simulink model "pfb_fir_test"  (Simulink 7.2)
settings: Solver=VariableStepDiscrete  StartTime=0.0  StopTime=500  RelTol=1e-3
undefined symbols (not defined in the file or in its folder): pfb_coeff_gen_calc
libraries: xbsIndex_r4 x240, casper_library_delays x20, casper_library_misc x18
(part 1 of 4)
settings Model: Creator=User  LastModifiedBy=root
settings OptimizationCC: InitFltsAndDblsToZero=on
settings DebuggingCC: SaveWithDisabledLinksMsg=none  SaveWithParameterizedLinksMsg=none

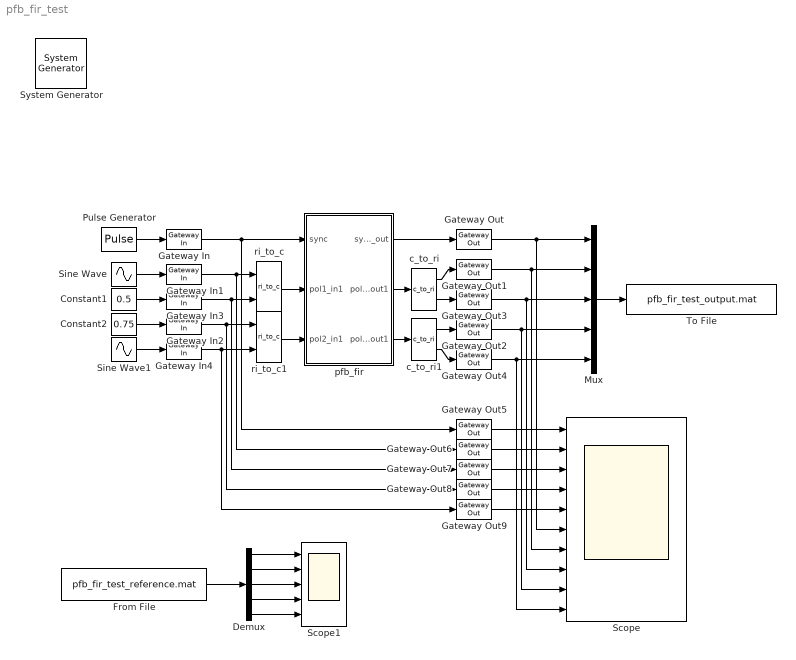
== system pfb_fir_test ==
  " System Generator" : xbsIndex_r4/ System Generator  Tag=genX  SystemSampleTime=-1  xilinxfamily=Virtex4  part=xc4vsx35  speed=-10  package=ff668  synthesis_tool=XST  clock_wrapper=Clock Enables  directory=./netlist  testbench=off  simulink_period=1  sysclk_period=100  dcm_input_clock_period=100  incr_netlist=off  trim_vbits=Everywhere in SubSystem  dbl_ovrd=According to Block Masks  core_generation=According to Block Masks  run_coregen=off  deprecated_control=off  eval_field=0  block_type=sysgen
      settings: block_version=10.1.1
  Constant1 : Constant  Value=0.5  OutDataType=sfix(16)  OutScaling=2^0
  Constant2 : Constant  Value=0.75  OutDataType=sfix(16)  OutScaling=2^0
  Demux : Demux  Outputs=5
  From File : FromFile  FileName=pfb_fir_test_reference.mat  SampleTime=1
  Gateway In : xbsIndex_r4/Gateway In  arith_type=Boolean  n_bits=16  bin_pt=14  quantization="Round  (unbiased: +/- Inf)"  overflow=Saturate  period=1  dbl_ovrd=off  timing_constraint=None  locs_specified=off  LOCs={}  hdl_port=on  block_type=gatewayin
      settings: infoedit="Gateway in block.  Converts inputs of type Simulink integer, double and fixed point to  Xilinx fixed point type.<P><P>Hardware notes:  In hardware these blocks become top level input ports."  block_version=10.1.1
  Gateway In{1..4} (4 alike) : xbsIndex_r4/Gateway In  arith_type="Signed  (2's comp)"  n_bits=12  bin_pt=11  quantization=Truncate  overflow=Wrap  period=1  dbl_ovrd=off  timing_constraint=None  locs_specified=off  LOCs={}  hdl_port=on  block_type=gatewayin
      settings: infoedit="Gateway in block.  Converts inputs of type Simulink integer, double and fixed point to  Xilinx fixed point type.<P><P>Hardware notes:  In hardware these blocks become top level input ports."  block_version=10.1.1
  Gateway Out{,1..9} (10 alike) : xbsIndex_r4/Gateway Out  hdl_port=on  timing_constraint=None  locs_specified=off  LOCs={}  block_type=gatewayout
      settings: infoedit="Gateway out block.  Converts Xilinx fixed point inputs into ouputs of type Simulink integer, double, or fixed point.<P><P>Hardware notes:  In hardware these blocks become top level output ports or are discarded, depending on how they are configured."  block_version=10.1.1
  Mux : Mux  Inputs=5
  Pulse Generator : DiscretePulseGenerator  Period=2^10  PhaseDelay=13
  Scope : Scope  NumInputPorts=10
      settings: YMin=-5~-5~-5~-5~-5~-5~-5~-5~-5~-5  YMax=5~5~5~5~5~5~5~5~5~5
  Scope1 : Scope  NumInputPorts=5
      settings: YMin=-5~-5~-5~-5~-5  YMax=5~5~5~5~5
  Sine Wave : Sin  SineType=Sample based  Amplitude=0.8  Samples=16  SampleTime=1  Offset=7
  Sine Wave1 : Sin  SineType=Sample based  Amplitude=0.8  Samples=8  SampleTime=1  Offset=7
  To File : ToFile  Filename=pfb_fir_test_output.mat  MatrixName=output
  c_to_ri : casper_library_misc/c_to_ri  SystemSampleTime=-1  n_bits=20  bin_pt=19
      settings: AttributesFormatString=20_19 r/i
  c_to_ri1 : casper_library_misc/c_to_ri  SystemSampleTime=-1  n_bits=20  bin_pt=19
      settings: AttributesFormatString=20_19 r/i
  pfb_fir : Subsystem  AncestorBlock=casper_library_pfbs/pfb_fir  mask(pfb_fir){PFBSize=6, TotalTaps=6, WindowType=nuttallwin, n_inputs=0, MakeBiplex=1, BitWidthIn=12, BitWidthOut=20, CoeffBitWidth=8, CoeffDistMem=1, add_latency=1, mult_latency=2, bram_latency=1, quantization=Round  (unbiased: +/- Inf), fwidth=0.75, specify_mult=off, mult_spec=[2                                      2]}
      mask prompts: PFBSize "Size of PFB: (2^? pnts)"; TotalTaps "Total Number of Taps:"; WindowType "Windowing Function:"; n_inputs "Number of Simultaneous Inputs: (2^?)"; MakeBiplex "Make Biplex"; BitWidthIn "Input Bitwidth:"; BitWidthOut "Output Bitwidth:"; CoeffBitWidth "Coefficient Bitwidth:"; CoeffDistMem "Use Distributed Memory for Coeffs"; add_latency "Add Latency"; mult_latency "Mult Latency"; bram_latency "BRAM Latency"; quantization "Quantization Behavior"; fwidth "Bin Width Scaling (normal=1)"; specify_mult "Specify multiplier use (behavioral if not specified)"; mult_spec "Multiplier specification (0=core, 1=embedded, 2=behavioural) (left=1st tap)"
      mask init:
      | pfb_fir_init(gcb, ...
      |     'PFBSize', PFBSize, ...
      |     'TotalTaps', TotalTaps, ...
      |     'WindowType', WindowType, ...
      |     'n_inputs', n_inputs, ...
      |     'MakeBiplex', MakeBiplex, ...
      |     'BitWidthIn', BitWidthIn, ...
      |     'BitWidthOut', BitWidthOut, ...
      |     'CoeffBitWidth', CoeffBitWidth, ...
      |     'CoeffDistMem', CoeffDistMem, ...
      |     'add_latency', add_latency, ...
      |     'mult_latency', mult_latency, ...
      |     'bram_latency', bram_latency, ...
      |     'quantization', quantization, ...
      |     'fwidth', fwidth,...
      |     'specify_mult', specify_mult,...
      |     'mult_spec', mult_spec);
      settings: AttributesFormatString=|
      | taps=6, add_latency=1
      | max scale 0.696
      mask Help: eval('xlWeb(''http://casper.berkeley.edu/wiki/Pfb_fir'')')
      mask StyleString: edit,edit,popup(bartlett|barthannwin|blackman|blackmanharris|bohamwin|chebwin|flattopwin|gausswin|hamming|hann|kaiser|nuttallwin|parzenwin|rectwin|tukeywin|triang|userwindow),edit,edit,edit,edit,edit,edit,edit,edit,edit,popup(Truncate|Round  (unbiased: +/- Inf)|Round  (unbiased: Even Values)),edit,checkbox,edit
      mask CallbackString:
      | |%num_taps = eval(get_param(gcb, 'TotalTaps'));
      | %old_vec = eval(get_param(gcb, 'mult_spec'));
      | 
      | %vec = 2.*ones(1,num_taps);
      | %old_size = length(old_vec);
      | 
      | %if(old_size <= num_taps),
      | %   new_size = old_size;
      | %else,
      | %    new_size = num_taps;
      | %end
      | 
      | %for n = 1:new_size, vec(n) = old_vec(n); end
      | %set_param(gcb, 'mult_spec', mat2str(vec));||||||||||||%num_taps = eval(get_param(gcb, 'TotalTaps'));
      | %old_vec = eval(get_param(gcb, 'mult_spec'));
      | 
      | %vec = 2.*ones(1,num_taps);
      | %old_size = length(old_vec);
      | 
      | %if(old_size <= num_taps),
      | %    new_size = old_size;
      | %else,
      | %    new_size = num_taps;
      | %end
      | 
      | %for n = 1:new_size, vec(n) = old_vec(n); end
      | %set_param(gcb, 'mult_spec', mat2str(vec));|%specify_mult = get_param(gcb,'specify_mult');
      | %if( strcmp(specify_mult,'off')),
      | %    set_param(gcb, 'MaskEnables', {'on','on','on','on','on','on','on','on','on','on','on','on','on','on','on','off'});
      | %else
      | %    set_param(gcb, 'MaskEnables', {'on','on','on','on','on','on','on','on','on','on','on','on','on','on','on','on'});
      | %end
      | 
      | |%specify_mult = get_param(gcb,'specify_mult');
      | %if( strcmp(specify_mult,'off')),
      | %    set_param(gcb, 'MaskEnables', {'on','on','on','on','on','on','on','on','on','on','on','on','on','on','on','off'});
      | %else
      | %    set_param(gcb, 'MaskEnables', {'on','on','on','on','on','on','on','on','on','on','on','on','on','on','on','on'});
      | %end
  ri_to_c : casper_library_misc/ri_to_c  SystemSampleTime=-1
  ri_to_c1 : casper_library_misc/ri_to_c  SystemSampleTime=-1
  wires:
  Pulse Generator/1 -> Gateway In/1
  Gateway In/1 -> Gateway Out5/1, pfb_fir/1(sync)
  Sine Wave/1 -> Gateway In1/1
  Constant2/1 -> Gateway In2/1
  pfb_fir/1(sync_out) -> Gateway Out/1
  Constant1/1 -> Gateway In3/1
  Sine Wave1/1 -> Gateway In4/1
  Gateway In1/1 -> ri_to_c/1, Gateway Out6/1
  Gateway In3/1 -> ri_to_c/2, Gateway Out7/1
  Gateway In2/1 -> ri_to_c1/1, Gateway Out8/1
  Gateway In4/1 -> ri_to_c1/2, Gateway Out9/1
  ri_to_c/1 -> pfb_fir/2(pol1_in1)
  ri_to_c1/1 -> pfb_fir/3(pol2_in1)
  pfb_fir/2(pol1_out1) -> c_to_ri/1
  c_to_ri/1 -> Gateway Out1/1
  c_to_ri/2 -> Gateway Out3/1
  pfb_fir/3(pol2_out1) -> c_to_ri1/1
  c_to_ri1/1 -> Gateway Out2/1
  c_to_ri1/2 -> Gateway Out4/1
  Gateway Out5/1 -> Scope/1
  Gateway Out6/1 -> Scope/2
  Gateway Out7/1 -> Scope/3
  Gateway Out8/1 -> Scope/4
  Gateway Out9/1 -> Scope/5
  Gateway Out/1 -> Scope/6, Mux/1
  Gateway Out1/1 -> Scope/7, Mux/2
  Gateway Out3/1 -> Scope/8, Mux/3
  Gateway Out2/1 -> Scope/9, Mux/4
  Gateway Out4/1 -> Scope/10, Mux/5
  Mux/1 -> To File/1
  From File/1 -> Demux/1
  Demux/1 -> Scope1/1
  Demux/2 -> Scope1/2
  Demux/3 -> Scope1/3
  Demux/4 -> Scope1/4
  Demux/5 -> Scope1/5

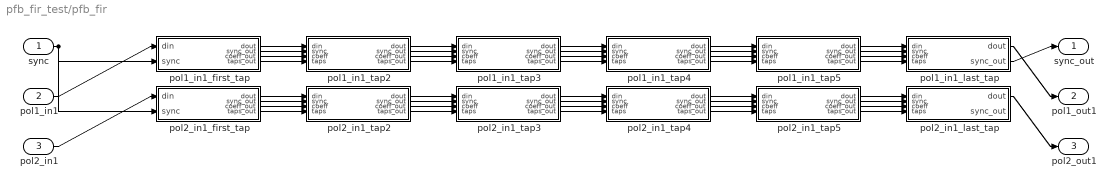
== system pfb_fir_test/pfb_fir ==
  sync : Inport
  pol1_in1 : Inport  Port=2
  pol2_in1 : Inport  Port=3
  pol1_in1_first_tap : Subsystem  AncestorBlock=casper_library_pfbs/first_tap  mask(first_tap){nput=0, PFBSize=6, CoeffBitWidth=8, TotalTaps=6, BitWidthIn=12, CoeffDistMem=1, WindowType=nuttallwin, mult_latency=2, bram_latency=1, n_inputs=0, fwidth=0.75, use_hdl=on, use_embedded=off}
      mask prompts: nput "This is input number:"; PFBSize "Size of PFB: (2^? pnts)"; CoeffBitWidth "Bitwidth of Coefficients:"; TotalTaps "Total Number of Taps:"; BitWidthIn "Input Bitwidth:"; CoeffDistMem "Implement Coeff Gen in Distributed Memory:"; WindowType "Windowing Function:"; mult_latency "Mult Latency"; bram_latency "BRAM Latency"; n_inputs "Number of Simultaneous Inputs: (2^?)"; fwidth "Bit Width (normal=1)"; use_hdl "Use behavioral HDL for multlipliers"; use_embedded "Use embedded multipliers"
      mask init:
      | first_tap_init(gcb,...
      |     'nput', nput,...
      |     'PFBSize', PFBSize,...
      |     'CoeffBitWidth', CoeffBitWidth,...
      |     'TotalTaps', TotalTaps,...
      |     'BitWidthIn', BitWidthIn,...
      |     'CoeffDistMem', CoeffDistMem,...
      |     'WindowType', WindowType,...
      |     'mult_latency', mult_latency,...
      |     'bram_latency', bram_latency,...
      |     'n_inputs', n_inputs,...
      |     'fwidth', fwidth,...
      |     'use_hdl', use_hdl,...
      |     'use_embedded', use_embedded);
      settings: AttributesFormatString=input=0, taps=6
      mask StyleString: edit,edit,edit,edit,edit,edit,popup(bartlett|barthannwin|blackman|blackmanharris|bohamwin|chebwin|flattopwin|gausswin|hamming|hann|kaiser|nuttallwin|parzenwin|rectwin|tukeywin|triang),edit,edit,edit,edit,checkbox,checkbox
      mask CallbackString:
      | |||||||||||use_hdl = get_param(gcb,'use_hdl');
      | if( strcmp(use_hdl,'on')),
      |     set_param(gcb, 'use_embedded','off');
      |     set_param(gcb, 'MaskVisibilities',{'on','on','on','on','on','on','on','on','on','on','on','on','off'});
      | else,
      |     set_param(gcb, 'MaskVisibilities',{'on','on','on','on','on','on','on','on','on','on','on','on','on'});
      | end
      | |
  pol1_in1_last_tap : Subsystem  AncestorBlock=casper_library_pfbs/last_tap  mask(last_tap){TotalTaps=6, BitWidthIn=12, BitWidthOut=20, CoeffBitWidth=8, add_latency=1, mult_latency=2, quantization=Round  (unbiased: +/- Inf), use_hdl=on, use_embedded=off}
      mask prompts: TotalTaps "Total Number of Taps:"; BitWidthIn "Input Bitwidth:"; BitWidthOut "Output Bitwidth:"; CoeffBitWidth "Coeff Bitwidth:"; add_latency "Add Latency"; mult_latency "Mult Latency"; quantization "Quantization Behavior"; use_hdl "Use behavioral HDL for multlipliers"; use_embedded "Use embedded multipliers"
      mask init:
      | last_tap_init(gcb,...
      |     'TotalTaps', TotalTaps,...
      |     'BitWidthIn', BitWidthIn,...
      |     'BitWidthOut', BitWidthOut,...
      |     'CoeffBitWidth', CoeffBitWidth,...
      |     'add_latency', add_latency,...
      |     'mult_latency', mult_latency,...
      |     'quantization', quantization,...
      |     'use_hdl', use_hdl,...
      |     'use_embedded', use_embedded);
      settings: AttributesFormatString=taps=6
      mask StyleString: edit,edit,edit,edit,edit,edit,popup(Truncate|Round  (unbiased: +/- Inf)|Round  (unbiased: Even Values)),checkbox,checkbox
      mask CallbackString:
      | |||||||use_hdl = get_param(gcb,'use_hdl');
      | if( strcmp(use_hdl,'on')),
      |     set_param(gcb, 'use_embedded','off');
      |     set_param(gcb, 'MaskVisibilities',{'on','on','on','on','on','on','on','on','off'});
      | else,
      |     set_param(gcb, 'MaskVisibilities',{'on','on','on','on','on','on','on','on','on'});
      | end
      | |
  pol1_in1_tap2 : Subsystem  AncestorBlock=casper_library_pfbs/tap  mask(tap){mult_latency=2, coeff_width=8, coeff_frac_width=7, delay=64, data_width=12, bram_latency=1, use_hdl=on, use_embedded=off}
      mask prompts: mult_latency "Multiplier Latency"; coeff_width "Coefficient Bit Width In"; coeff_frac_width "Coefficient Fractional Bits"; delay "Data/Sync Delay"; data_width "Data Bit Width In"; bram_latency "BRAM Latency"; use_hdl "Use behavioral HDL for multlipliers"; use_embedded "Use embedded multipliers"
      mask init:
      | use_hdl = get_param(gcb,'use_hdl');
      | use_embedded = get_param(gcb,'use_embedded');
      | set_param(gcb,'LinkStatus','inactive');
      | 
      | set_param([gcb,'/Mult'],'use_embedded',use_embedded);
      | set_param([gcb,'/Mult'],'use_behavioral_HDL',use_hdl);
      | set_param([gcb,'/Mult1'],'use_embedded',use_embedded);
      | set_param([gcb,'/Mult1'],'use_behavioral_HDL',use_hdl);
      mask CallbackString:
      | ||||||use_hdl = get_param(gcb,'use_hdl');
      | if( strcmp(use_hdl,'on')),
      |     set_param(gcb, 'use_embedded','off');
      |     set_param(gcb, 'MaskVisibilities',{'on','on','on','on','on','on','on','off'});
      | else,
      |     set_param(gcb, 'MaskVisibilities',{'on','on','on','on','on','on','on','on'});
      | end
      | |
  pol1_in1_tap3 : Subsystem  AncestorBlock=casper_library_pfbs/tap  mask(tap){mult_latency=2, coeff_width=8, coeff_frac_width=7, delay=64, data_width=12, bram_latency=1, use_hdl=on, use_embedded=off}
      mask prompts: mult_latency "Multiplier Latency"; coeff_width "Coefficient Bit Width In"; coeff_frac_width "Coefficient Fractional Bits"; delay "Data/Sync Delay"; data_width "Data Bit Width In"; bram_latency "BRAM Latency"; use_hdl "Use behavioral HDL for multlipliers"; use_embedded "Use embedded multipliers"
      mask init: same as pfb_fir_test/pfb_fir/pol1_in1_tap2
      mask CallbackString:
      | ||||||use_hdl = get_param(gcb,'use_hdl');
      | if( strcmp(use_hdl,'on')),
      |     set_param(gcb, 'use_embedded','off');
      |     set_param(gcb, 'MaskVisibilities',{'on','on','on','on','on','on','on','off'});
      | else,
      |     set_param(gcb, 'MaskVisibilities',{'on','on','on','on','on','on','on','on'});
      | end
      | |
  pol1_in1_tap4 : Subsystem  AncestorBlock=casper_library_pfbs/tap  mask(tap){mult_latency=2, coeff_width=8, coeff_frac_width=7, delay=64, data_width=12, bram_latency=1, use_hdl=on, use_embedded=off}
      mask prompts: mult_latency "Multiplier Latency"; coeff_width "Coefficient Bit Width In"; coeff_frac_width "Coefficient Fractional Bits"; delay "Data/Sync Delay"; data_width "Data Bit Width In"; bram_latency "BRAM Latency"; use_hdl "Use behavioral HDL for multlipliers"; use_embedded "Use embedded multipliers"
      mask init: same as pfb_fir_test/pfb_fir/pol1_in1_tap2
      mask CallbackString:
      | ||||||use_hdl = get_param(gcb,'use_hdl');
      | if( strcmp(use_hdl,'on')),
      |     set_param(gcb, 'use_embedded','off');
      |     set_param(gcb, 'MaskVisibilities',{'on','on','on','on','on','on','on','off'});
      | else,
      |     set_param(gcb, 'MaskVisibilities',{'on','on','on','on','on','on','on','on'});
      | end
      | |
  pol1_in1_tap5 : Subsystem  AncestorBlock=casper_library_pfbs/tap  mask(tap){mult_latency=2, coeff_width=8, coeff_frac_width=7, delay=64, data_width=12, bram_latency=1, use_hdl=on, use_embedded=off}
      mask prompts: mult_latency "Multiplier Latency"; coeff_width "Coefficient Bit Width In"; coeff_frac_width "Coefficient Fractional Bits"; delay "Data/Sync Delay"; data_width "Data Bit Width In"; bram_latency "BRAM Latency"; use_hdl "Use behavioral HDL for multlipliers"; use_embedded "Use embedded multipliers"
      mask init: same as pfb_fir_test/pfb_fir/pol1_in1_tap2
      mask CallbackString:
      | ||||||use_hdl = get_param(gcb,'use_hdl');
      | if( strcmp(use_hdl,'on')),
      |     set_param(gcb, 'use_embedded','off');
      |     set_param(gcb, 'MaskVisibilities',{'on','on','on','on','on','on','on','off'});
      | else,
      |     set_param(gcb, 'MaskVisibilities',{'on','on','on','on','on','on','on','on'});
      | end
      | |
  pol2_in1_first_tap : Subsystem  AncestorBlock=casper_library_pfbs/first_tap  mask(first_tap){nput=0, PFBSize=6, CoeffBitWidth=8, TotalTaps=6, BitWidthIn=12, CoeffDistMem=1, WindowType=nuttallwin, mult_latency=2, bram_latency=1, n_inputs=0, fwidth=0.75, use_hdl=on, use_embedded=off}
      mask prompts: nput "This is input number:"; PFBSize "Size of PFB: (2^? pnts)"; CoeffBitWidth "Bitwidth of Coefficients:"; TotalTaps "Total Number of Taps:"; BitWidthIn "Input Bitwidth:"; CoeffDistMem "Implement Coeff Gen in Distributed Memory:"; WindowType "Windowing Function:"; mult_latency "Mult Latency"; bram_latency "BRAM Latency"; n_inputs "Number of Simultaneous Inputs: (2^?)"; fwidth "Bit Width (normal=1)"; use_hdl "Use behavioral HDL for multlipliers"; use_embedded "Use embedded multipliers"
      mask init: same as pfb_fir_test/pfb_fir/pol1_in1_first_tap
      settings: AttributesFormatString=input=0, taps=6
      mask StyleString: edit,edit,edit,edit,edit,edit,popup(bartlett|barthannwin|blackman|blackmanharris|bohamwin|chebwin|flattopwin|gausswin|hamming|hann|kaiser|nuttallwin|parzenwin|rectwin|tukeywin|triang),edit,edit,edit,edit,checkbox,checkbox
      mask CallbackString:
      | |||||||||||use_hdl = get_param(gcb,'use_hdl');
      | if( strcmp(use_hdl,'on')),
      |     set_param(gcb, 'use_embedded','off');
      |     set_param(gcb, 'MaskVisibilities',{'on','on','on','on','on','on','on','on','on','on','on','on','off'});
      | else,
      |     set_param(gcb, 'MaskVisibilities',{'on','on','on','on','on','on','on','on','on','on','on','on','on'});
      | end
      | |
  pol2_in1_last_tap : Subsystem  AncestorBlock=casper_library_pfbs/last_tap  mask(last_tap){TotalTaps=6, BitWidthIn=12, BitWidthOut=20, CoeffBitWidth=8, add_latency=1, mult_latency=2, quantization=Round  (unbiased: +/- Inf), use_hdl=on, use_embedded=off}
      mask prompts: TotalTaps "Total Number of Taps:"; BitWidthIn "Input Bitwidth:"; BitWidthOut "Output Bitwidth:"; CoeffBitWidth "Coeff Bitwidth:"; add_latency "Add Latency"; mult_latency "Mult Latency"; quantization "Quantization Behavior"; use_hdl "Use behavioral HDL for multlipliers"; use_embedded "Use embedded multipliers"
      mask init: same as pfb_fir_test/pfb_fir/pol1_in1_last_tap
      settings: AttributesFormatString=taps=6
      mask StyleString: edit,edit,edit,edit,edit,edit,popup(Truncate|Round  (unbiased: +/- Inf)|Round  (unbiased: Even Values)),checkbox,checkbox
      mask CallbackString:
      | |||||||use_hdl = get_param(gcb,'use_hdl');
      | if( strcmp(use_hdl,'on')),
      |     set_param(gcb, 'use_embedded','off');
      |     set_param(gcb, 'MaskVisibilities',{'on','on','on','on','on','on','on','on','off'});
      | else,
      |     set_param(gcb, 'MaskVisibilities',{'on','on','on','on','on','on','on','on','on'});
      | end
      | |
  pol2_in1_tap2 : Subsystem  AncestorBlock=casper_library_pfbs/tap  mask(tap){mult_latency=2, coeff_width=8, coeff_frac_width=7, delay=64, data_width=12, bram_latency=1, use_hdl=on, use_embedded=off}
      mask prompts: mult_latency "Multiplier Latency"; coeff_width "Coefficient Bit Width In"; coeff_frac_width "Coefficient Fractional Bits"; delay "Data/Sync Delay"; data_width "Data Bit Width In"; bram_latency "BRAM Latency"; use_hdl "Use behavioral HDL for multlipliers"; use_embedded "Use embedded multipliers"
      mask init: same as pfb_fir_test/pfb_fir/pol1_in1_tap2
      mask CallbackString:
      | ||||||use_hdl = get_param(gcb,'use_hdl');
      | if( strcmp(use_hdl,'on')),
      |     set_param(gcb, 'use_embedded','off');
      |     set_param(gcb, 'MaskVisibilities',{'on','on','on','on','on','on','on','off'});
      | else,
      |     set_param(gcb, 'MaskVisibilities',{'on','on','on','on','on','on','on','on'});
      | end
      | |
  pol2_in1_tap3 : Subsystem  AncestorBlock=casper_library_pfbs/tap  mask(tap){mult_latency=2, coeff_width=8, coeff_frac_width=7, delay=64, data_width=12, bram_latency=1, use_hdl=on, use_embedded=off}
      mask prompts: mult_latency "Multiplier Latency"; coeff_width "Coefficient Bit Width In"; coeff_frac_width "Coefficient Fractional Bits"; delay "Data/Sync Delay"; data_width "Data Bit Width In"; bram_latency "BRAM Latency"; use_hdl "Use behavioral HDL for multlipliers"; use_embedded "Use embedded multipliers"
      mask init: same as pfb_fir_test/pfb_fir/pol1_in1_tap2
      mask CallbackString:
      | ||||||use_hdl = get_param(gcb,'use_hdl');
      | if( strcmp(use_hdl,'on')),
      |     set_param(gcb, 'use_embedded','off');
      |     set_param(gcb, 'MaskVisibilities',{'on','on','on','on','on','on','on','off'});
      | else,
      |     set_param(gcb, 'MaskVisibilities',{'on','on','on','on','on','on','on','on'});
      | end
      | |
  pol2_in1_tap4 : Subsystem  AncestorBlock=casper_library_pfbs/tap  mask(tap){mult_latency=2, coeff_width=8, coeff_frac_width=7, delay=64, data_width=12, bram_latency=1, use_hdl=on, use_embedded=off}
      mask prompts: mult_latency "Multiplier Latency"; coeff_width "Coefficient Bit Width In"; coeff_frac_width "Coefficient Fractional Bits"; delay "Data/Sync Delay"; data_width "Data Bit Width In"; bram_latency "BRAM Latency"; use_hdl "Use behavioral HDL for multlipliers"; use_embedded "Use embedded multipliers"
      mask init: same as pfb_fir_test/pfb_fir/pol1_in1_tap2
      mask CallbackString:
      | ||||||use_hdl = get_param(gcb,'use_hdl');
      | if( strcmp(use_hdl,'on')),
      |     set_param(gcb, 'use_embedded','off');
      |     set_param(gcb, 'MaskVisibilities',{'on','on','on','on','on','on','on','off'});
      | else,
      |     set_param(gcb, 'MaskVisibilities',{'on','on','on','on','on','on','on','on'});
      | end
      | |
  pol2_in1_tap5 : Subsystem  AncestorBlock=casper_library_pfbs/tap  mask(tap){mult_latency=2, coeff_width=8, coeff_frac_width=7, delay=64, data_width=12, bram_latency=1, use_hdl=on, use_embedded=off}
      mask prompts: mult_latency "Multiplier Latency"; coeff_width "Coefficient Bit Width In"; coeff_frac_width "Coefficient Fractional Bits"; delay "Data/Sync Delay"; data_width "Data Bit Width In"; bram_latency "BRAM Latency"; use_hdl "Use behavioral HDL for multlipliers"; use_embedded "Use embedded multipliers"
      mask init: same as pfb_fir_test/pfb_fir/pol1_in1_tap2
      mask CallbackString:
      | ||||||use_hdl = get_param(gcb,'use_hdl');
      | if( strcmp(use_hdl,'on')),
      |     set_param(gcb, 'use_embedded','off');
      |     set_param(gcb, 'MaskVisibilities',{'on','on','on','on','on','on','on','off'});
      | else,
      |     set_param(gcb, 'MaskVisibilities',{'on','on','on','on','on','on','on','on'});
      | end
      | |
  sync_out : Outport
  pol1_out1 : Outport  Port=2
  pol2_out1 : Outport  Port=3
  wires:
  pol1_in1/1 -> pol1_in1_first_tap/1(din)
  sync/1 -> pol1_in1_first_tap/2(sync), pol2_in1_first_tap/2(sync)
  pol1_in1_first_tap/1(dout) -> pol1_in1_tap2/1(din)
  pol1_in1_first_tap/2(sync_out) -> pol1_in1_tap2/2(sync)
  pol1_in1_first_tap/3(coeff_out) -> pol1_in1_tap2/3(coeff)
  pol1_in1_first_tap/4(taps_out) -> pol1_in1_tap2/4(taps)
  pol1_in1_tap2/1(dout) -> pol1_in1_tap3/1(din)
  pol1_in1_tap2/2(sync_out) -> pol1_in1_tap3/2(sync)
  pol1_in1_tap2/3(coeff_out) -> pol1_in1_tap3/3(coeff)
  pol1_in1_tap2/4(taps_out) -> pol1_in1_tap3/4(taps)
  pol1_in1_tap3/1(dout) -> pol1_in1_tap4/1(din)
  pol1_in1_tap3/2(sync_out) -> pol1_in1_tap4/2(sync)
  pol1_in1_tap3/3(coeff_out) -> pol1_in1_tap4/3(coeff)
  pol1_in1_tap3/4(taps_out) -> pol1_in1_tap4/4(taps)
  pol1_in1_tap4/1(dout) -> pol1_in1_tap5/1(din)
  pol1_in1_tap4/2(sync_out) -> pol1_in1_tap5/2(sync)
  pol1_in1_tap4/3(coeff_out) -> pol1_in1_tap5/3(coeff)
  pol1_in1_tap4/4(taps_out) -> pol1_in1_tap5/4(taps)
  pol1_in1_tap5/1(dout) -> pol1_in1_last_tap/1(din)
  pol1_in1_tap5/2(sync_out) -> pol1_in1_last_tap/2(sync)
  pol1_in1_tap5/3(coeff_out) -> pol1_in1_last_tap/3(coeff)
  pol1_in1_tap5/4(taps_out) -> pol1_in1_last_tap/4(taps)
  pol1_in1_last_tap/1(dout) -> pol1_out1/1
  pol1_in1_last_tap/2(sync_out) -> sync_out/1
  pol2_in1/1 -> pol2_in1_first_tap/1(din)
  pol2_in1_first_tap/1(dout) -> pol2_in1_tap2/1(din)
  pol2_in1_first_tap/2(sync_out) -> pol2_in1_tap2/2(sync)
  pol2_in1_first_tap/3(coeff_out) -> pol2_in1_tap2/3(coeff)
  pol2_in1_first_tap/4(taps_out) -> pol2_in1_tap2/4(taps)
  pol2_in1_tap2/1(dout) -> pol2_in1_tap3/1(din)
  pol2_in1_tap2/2(sync_out) -> pol2_in1_tap3/2(sync)
  pol2_in1_tap2/3(coeff_out) -> pol2_in1_tap3/3(coeff)
  pol2_in1_tap2/4(taps_out) -> pol2_in1_tap3/4(taps)
  pol2_in1_tap3/1(dout) -> pol2_in1_tap4/1(din)
  pol2_in1_tap3/2(sync_out) -> pol2_in1_tap4/2(sync)
  pol2_in1_tap3/3(coeff_out) -> pol2_in1_tap4/3(coeff)
  pol2_in1_tap3/4(taps_out) -> pol2_in1_tap4/4(taps)
  pol2_in1_tap4/1(dout) -> pol2_in1_tap5/1(din)
  pol2_in1_tap4/2(sync_out) -> pol2_in1_tap5/2(sync)
  pol2_in1_tap4/3(coeff_out) -> pol2_in1_tap5/3(coeff)
  pol2_in1_tap4/4(taps_out) -> pol2_in1_tap5/4(taps)
  pol2_in1_tap5/1(dout) -> pol2_in1_last_tap/1(din)
  pol2_in1_tap5/2(sync_out) -> pol2_in1_last_tap/2(sync)
  pol2_in1_tap5/3(coeff_out) -> pol2_in1_last_tap/3(coeff)
  pol2_in1_tap5/4(taps_out) -> pol2_in1_last_tap/4(taps)
  pol2_in1_last_tap/1(dout) -> pol2_out1/1

== system pfb_fir_test/pfb_fir/pol1_in1_first_tap ==
  din : Inport  OutDataType=sfix(16)  OutScaling=2^0
  sync : Inport  Port=2  OutDataType=sfix(16)  OutScaling=2^0
  Mult : xbsIndex_r4/Mult  precision=Full  arith_type="Signed  (2's comp)"  n_bits=8  bin_pt=2  quantization=Truncate  overflow=Wrap  en=off  latency=mult_latency  dbl_ovrd=off  use_behavioral_HDL=on  opt=Speed  use_embedded=off  optimum_pipeline=off  pipeline=on  use_rpm=on  placement_style=Rectangular shape  block_type=mult
      settings: infoedit=Hardware notes: To use the internal pipeline stage of the dedicated multiplier you must select 'Pipeline for maximum performance'.  xl_area=[0, 0, 0, 0, 0, 0, 0]  block_version=9.1.01
  Mult1 : xbsIndex_r4/Mult  precision=Full  arith_type="Signed  (2's comp)"  n_bits=8  bin_pt=2  quantization=Truncate  overflow=Wrap  en=off  latency=mult_latency  dbl_ovrd=off  use_behavioral_HDL=on  opt=Speed  use_embedded=off  optimum_pipeline=off  pipeline=on  use_rpm=on  placement_style=Rectangular shape  block_type=mult
      settings: infoedit=Hardware notes: To use the internal pipeline stage of the dedicated multiplier you must select 'Pipeline for maximum performance'.  xl_area=[0, 0, 0, 0, 0, 0, 0]  block_version=9.1.01
  Reinterpret : xbsIndex_r4/Reinterpret  force_arith_type=on  arith_type="Signed  (2's comp)"  force_bin_pt=on  bin_pt=CoeffBitWidth - 1  block_type=reinterpret
      settings: infoedit="Changes signal type without altering the binary representation.   You can changed the signal between signed and unsigned, and relocate the binary point.<P><P>Hardware notes: In hardware this block costs nothing.<P><P>Example:  Suppose the input is 6 bits wide, signed, with 2 fractional bits, and the output is forced to unsigned with 0 fractional bits.  Then an input of -2.0 (1110.00 in binary 2's complement) becomes an output of 56 (111000 in binary)."  block_version=9.1.01
  Slice : xbsIndex_r4/Slice  nbits=CoeffBitWidth  boolean_output=off  mode=Lower Bit Location + Width  bit1=0  base1=MSB of Input  bit0=0  base0=LSB of Input  dbl_ovrd=off  block_type=slice
      settings: infoedit="Extracts a given range of bits from each input sample and presents it at the output.  The output type is ordinarily unsigned with binary point at zero, but can be Boolean when the slice is one bit wide.<P><P>Hardware notes: In hardware this block costs nothing."  block_version=9.1.01
  Slice1 : xbsIndex_r4/Slice  nbits=CoeffBitWidth * (TotalTaps - 1)  boolean_output=off  mode=Two Bit Locations  bit1=0  base1=MSB of Input  bit0=CoeffBitWidth  base0=LSB of Input  dbl_ovrd=off  block_type=slice
      settings: infoedit="Extracts a given range of bits from each input sample and presents it at the output.  The output type is ordinarily unsigned with binary point at zero, but can be Boolean when the slice is one bit wide.<P><P>Hardware notes: In hardware this block costs nothing."  block_version=9.1.01
  c_to_ri : casper_library_misc/c_to_ri  SystemSampleTime=-1  n_bits=BitWidthIn  bin_pt=BitWidthIn-1
      settings: AttributesFormatString=12_11 r/i
  delay_bram : casper_library_delays/delay_bram  SystemSampleTime=-1  DelayLen=2^(PFBSize-n_inputs)  bram_latency=bram_latency  use_dsp48=off
  pfb_coeff_gen : Subsystem  AncestorBlock=casper_library_pfbs/pfb_coeff_gen  mask(pfb_coeff_gen){PFBSize=6, CoeffBitWidth=8, TotalTaps=6, CoeffDistMem=1, WindowType=nuttallwin, bram_latency=1, n_inputs=0, nput=0, fwidth=0.75}
      mask prompts: PFBSize "Size of PFB: (2^? pnts)"; CoeffBitWidth "Bitwidth of Coefficients:"; TotalTaps "Total Number of Taps:"; CoeffDistMem "Implement Coeff Gen in Distributed Memory"; WindowType "Windowing Function:"; bram_latency "BRAM Latency"; n_inputs "Number of Simultaneous Inputs: (2^?)"; nput "This is input number:"; fwidth "Bin Width (normal=1)"
      mask init:
      | pfb_coeff_gen_init(gcb, ...
      |     'PFBSize', PFBSize, ...
      |     'CoeffBitWidth', CoeffBitWidth, ...
      |     'TotalTaps', TotalTaps, ...
      |     'CoeffDistMem', CoeffDistMem, ...
      |     'WindowType', WindowType, ...
      |     'bram_latency', bram_latency, ...
      |     'n_inputs', n_inputs, ...
      |     'nput', nput, ...
      |     'fwidth', fwidth);
      settings: AttributesFormatString=PFBSize=6, n_inputs=0, taps=6
  ri_to_c : Subsystem
  sync_delay : casper_library_delays/sync_delay  SystemSampleTime=-1  DelayLen=2^(PFBSize-n_inputs)
  dout : Outport  OutDataType=sfix(16)  OutScaling=2^0
  sync_out : Outport  Port=2  OutDataType=sfix(16)  OutScaling=2^0
  coeff_out : Outport  Port=3  OutDataType=sfix(16)  OutScaling=2^0
  taps_out : Outport  Port=4  OutDataType=sfix(16)  OutScaling=2^0
  wires:
  ri_to_c/1(c) -> taps_out/1
  Mult/1 -> ri_to_c/2(im)
  Mult1/1 -> ri_to_c/1(re)
  c_to_ri/2 -> Mult/1
  c_to_ri/1 -> Mult1/1
  pfb_coeff_gen/3(coeff) -> Slice1/1, Slice/1
  pfb_coeff_gen/2(sync_out) -> sync_delay/1
  sync/1 -> pfb_coeff_gen/2(sync)
  pfb_coeff_gen/1(dout) -> delay_bram/1, c_to_ri/1
  din/1 -> pfb_coeff_gen/1(din)
  delay_bram/1 -> dout/1
  sync_delay/1 -> sync_out/1
  Slice1/1 -> coeff_out/1
  Slice/1 -> Reinterpret/1
  Reinterpret/1 -> Mult1/2, Mult/2

== system pfb_fir_test/pfb_fir/pol1_in1_last_tap ==
  din : Inport  OutDataType=sfix(16)  OutScaling=2^0
  sync : Inport  Port=2  OutDataType=sfix(16)  OutScaling=2^0
  coeff : Inport  Port=3  OutDataType=sfix(16)  OutScaling=2^0
  taps : Inport  Port=4  OutDataType=sfix(16)  OutScaling=2^0
  Concat : xbsIndex_r4/Concat  num_inputs=2  dbl_ovrd=off  block_type=concat
      settings: block_version=9.1.01
  Delay : xbsIndex_r4/Delay  en=off  latency=mult_latency  dbl_ovrd=off  reg_retiming=off  block_type=delay
      settings: xl_area=[0, 0, 0, 0, 0, 0, 0]  block_version=9.1.01
  Mult : xbsIndex_r4/Mult  precision=Full  arith_type="Signed  (2's comp)"  n_bits=8  bin_pt=2  quantization=Truncate  overflow=Wrap  en=off  latency=mult_latency  dbl_ovrd=off  use_behavioral_HDL=on  opt=Speed  use_embedded=off  optimum_pipeline=off  pipeline=on  use_rpm=on  placement_style=Rectangular shape  block_type=mult
      settings: infoedit=Hardware notes: To use the internal pipeline stage of the dedicated multiplier you must select 'Pipeline for maximum performance'.  xl_area=[0, 0, 0, 0, 0, 0, 0]  block_version=9.1.01
  Mult1 : xbsIndex_r4/Mult  precision=Full  arith_type="Signed  (2's comp)"  n_bits=8  bin_pt=2  quantization=Truncate  overflow=Wrap  en=off  latency=mult_latency  dbl_ovrd=off  use_behavioral_HDL=on  opt=Speed  use_embedded=off  optimum_pipeline=off  pipeline=on  use_rpm=on  placement_style=Rectangular shape  block_type=mult
      settings: infoedit=Hardware notes: To use the internal pipeline stage of the dedicated multiplier you must select 'Pipeline for maximum performance'.  xl_area=[0, 0, 0, 0, 0, 0, 0]  block_version=9.1.01
  Reinterpret : xbsIndex_r4/Reinterpret  force_arith_type=on  arith_type="Signed  (2's comp)"  force_bin_pt=on  bin_pt=CoeffBitWidth - 1  block_type=reinterpret
      settings: infoedit="Changes signal type without altering the binary representation.   You can changed the signal between signed and unsigned, and relocate the binary point.<P><P>Hardware notes: In hardware this block costs nothing.<P><P>Example:  Suppose the input is 6 bits wide, signed, with 2 fractional bits, and the output is forced to unsigned with 0 fractional bits.  Then an input of -2.0 (1110.00 in binary 2's complement) becomes an output of 56 (111000 in binary)."  block_version=9.1.01
  c_to_ri : casper_library_misc/c_to_ri  SystemSampleTime=-1  n_bits=BitWidthIn  bin_pt=BitWidthIn-1
      settings: AttributesFormatString=12_11 r/i
  pfb_add_tree : Subsystem  mask(pfb_add_tree){TotalTaps=6, BitWidthIn=12, BitWidthOut=20, CoeffBitWidth=8, add_latency=1, quantization=Round  (unbiased: +/- Inf)}
      mask prompts: TotalTaps "Total Number of Taps:"; BitWidthIn "Input Bitwidth:"; BitWidthOut "Output Bitwidth:"; CoeffBitWidth "Coeff Bitwidth:"; add_latency "Add Latency"; quantization "Quantization Behavior"
      mask init:
      | pfb_add_tree_init(gcb, ...
      |     'TotalTaps', TotalTaps, ...
      |     'BitWidthIn', BitWidthIn, ...
      |     'BitWidthOut', BitWidthOut, ...
      |     'CoeffBitWidth', CoeffBitWidth, ...
      |     'add_latency', add_latency, ...
      |     'quantization', quantization);
      settings: AttributesFormatString=taps=6, add_latency=1
      mask StyleString: edit,edit,edit,edit,edit,popup(Truncate|Round  (unbiased: +/- Inf)|Round  (unbiased: Even Values))
  ri_to_c : Subsystem
  dout : Outport  OutDataType=sfix(16)  OutScaling=2^0
  sync_out : Outport  Port=2  OutDataType=sfix(16)  OutScaling=2^0
  wires:
  Reinterpret/1 -> Mult/2, Mult1/2
  coeff/1 -> Reinterpret/1
  Concat/1 -> pfb_add_tree/1(din)
  taps/1 -> Concat/2
  sync/1 -> Delay/1
  pfb_add_tree/1(dout) -> dout/1
  pfb_add_tree/2(sync_out) -> sync_out/1
  Delay/1 -> pfb_add_tree/2(sync)
  c_to_ri/1 -> Mult1/1
  c_to_ri/2 -> Mult/1
  din/1 -> c_to_ri/1
  Mult1/1 -> ri_to_c/1(re)
  Mult/1 -> ri_to_c/2(im)
  ri_to_c/1(c) -> Concat/1

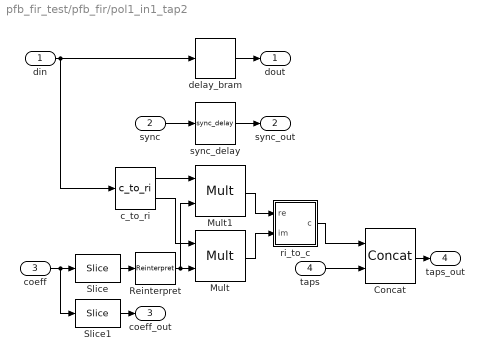
== system pfb_fir_test/pfb_fir/pol1_in1_tap2 ==
  din : Inport  OutDataType=sfix(16)  OutScaling=2^0
  sync : Inport  Port=2  OutDataType=sfix(16)  OutScaling=2^0
  coeff : Inport  Port=3  OutDataType=sfix(16)  OutScaling=2^0
  taps : Inport  Port=4  OutDataType=sfix(16)  OutScaling=2^0
  Concat : xbsIndex_r4/Concat  num_inputs=2  dbl_ovrd=off  block_type=concat
      settings: block_version=9.1.01
  Mult : xbsIndex_r4/Mult  precision=Full  arith_type="Signed  (2's comp)"  n_bits=8  bin_pt=2  quantization=Truncate  overflow=Wrap  en=off  latency=mult_latency  dbl_ovrd=off  use_behavioral_HDL=on  opt=Speed  use_embedded=off  optimum_pipeline=off  pipeline=on  use_rpm=on  placement_style=Rectangular shape  block_type=mult
      settings: infoedit=Hardware notes: To use the internal pipeline stage of the dedicated multiplier you must select 'Pipeline for maximum performance'.  xl_area=[0, 0, 0, 0, 0, 0, 0]  block_version=9.1.01
  Mult1 : xbsIndex_r4/Mult  precision=Full  arith_type="Signed  (2's comp)"  n_bits=8  bin_pt=2  quantization=Truncate  overflow=Wrap  en=off  latency=mult_latency  dbl_ovrd=off  use_behavioral_HDL=on  opt=Speed  use_embedded=off  optimum_pipeline=off  pipeline=on  use_rpm=on  placement_style=Rectangular shape  block_type=mult
      settings: infoedit=Hardware notes: To use the internal pipeline stage of the dedicated multiplier you must select 'Pipeline for maximum performance'.  xl_area=[0, 0, 0, 0, 0, 0, 0]  block_version=9.1.01
  Reinterpret : xbsIndex_r4/Reinterpret  force_arith_type=on  arith_type="Signed  (2's comp)"  force_bin_pt=on  bin_pt=coeff_frac_width  block_type=reinterpret
      settings: infoedit="Changes signal type without altering the binary representation.   You can changed the signal between signed and unsigned, and relocate the binary point.<P><P>Hardware notes: In hardware this block costs nothing.<P><P>Example:  Suppose the input is 6 bits wide, signed, with 2 fractional bits, and the output is forced to unsigned with 0 fractional bits.  Then an input of -2.0 (1110.00 in binary 2's complement) becomes an output of 56 (111000 in binary)."  block_version=9.1.01
  Slice : xbsIndex_r4/Slice  nbits=coeff_width  boolean_output=off  mode=Lower Bit Location + Width  bit1=0  base1=MSB of Input  bit0=0  base0=LSB of Input  dbl_ovrd=off  block_type=slice
      settings: infoedit="Extracts a given range of bits from each input sample and presents it at the output.  The output type is ordinarily unsigned with binary point at zero, but can be Boolean when the slice is one bit wide.<P><P>Hardware notes: In hardware this block costs nothing."  block_version=9.1.01
  Slice1 : xbsIndex_r4/Slice  nbits=0  boolean_output=off  mode=Two Bit Locations  bit1=0  base1=MSB of Input  bit0=coeff_width  base0=LSB of Input  dbl_ovrd=off  block_type=slice
      settings: infoedit="Extracts a given range of bits from each input sample and presents it at the output.  The output type is ordinarily unsigned with binary point at zero, but can be Boolean when the slice is one bit wide.<P><P>Hardware notes: In hardware this block costs nothing."  block_version=9.1.01
  c_to_ri : casper_library_misc/c_to_ri  SystemSampleTime=-1  n_bits=data_width  bin_pt=data_width-1
      settings: AttributesFormatString=12_11 r/i
  delay_bram : casper_library_delays/delay_bram  SystemSampleTime=-1  DelayLen=delay  bram_latency=bram_latency  use_dsp48=off
  ri_to_c : Subsystem
  sync_delay : casper_library_delays/sync_delay  SystemSampleTime=-1  DelayLen=delay
  dout : Outport  OutDataType=sfix(16)  OutScaling=2^0
  sync_out : Outport  Port=2  OutDataType=sfix(16)  OutScaling=2^0
  coeff_out : Outport  Port=3  OutDataType=sfix(16)  OutScaling=2^0
  taps_out : Outport  Port=4  OutDataType=sfix(16)  OutScaling=2^0
  wires:
  delay_bram/1 -> dout/1
  din/1 -> delay_bram/1, c_to_ri/1
  c_to_ri/2 -> Mult/1
  c_to_ri/1 -> Mult1/1
  ri_to_c/1(c) -> Concat/1
  Mult/1 -> ri_to_c/2(im)
  Mult1/1 -> ri_to_c/1(re)
  sync/1 -> sync_delay/1
  sync_delay/1 -> sync_out/1
  taps/1 -> Concat/2
  Concat/1 -> taps_out/1
  coeff/1 -> Slice/1, Slice1/1
  Slice1/1 -> coeff_out/1
  Slice/1 -> Reinterpret/1
  Reinterpret/1 -> Mult1/2, Mult/2

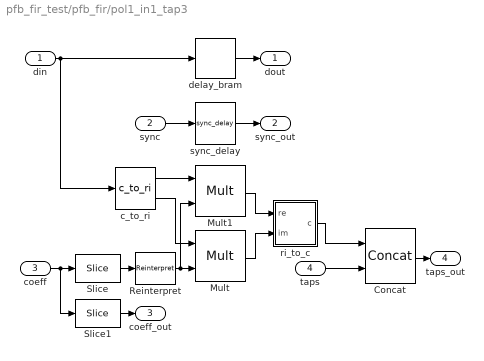
== system pfb_fir_test/pfb_fir/pol1_in1_tap3 ==
  din : Inport  OutDataType=sfix(16)  OutScaling=2^0
  sync : Inport  Port=2  OutDataType=sfix(16)  OutScaling=2^0
  coeff : Inport  Port=3  OutDataType=sfix(16)  OutScaling=2^0
  taps : Inport  Port=4  OutDataType=sfix(16)  OutScaling=2^0
  Concat : xbsIndex_r4/Concat  num_inputs=2  dbl_ovrd=off  block_type=concat
      settings: block_version=9.1.01
  Mult : xbsIndex_r4/Mult  precision=Full  arith_type="Signed  (2's comp)"  n_bits=8  bin_pt=2  quantization=Truncate  overflow=Wrap  en=off  latency=mult_latency  dbl_ovrd=off  use_behavioral_HDL=on  opt=Speed  use_embedded=off  optimum_pipeline=off  pipeline=on  use_rpm=on  placement_style=Rectangular shape  block_type=mult
      settings: infoedit=Hardware notes: To use the internal pipeline stage of the dedicated multiplier you must select 'Pipeline for maximum performance'.  xl_area=[0, 0, 0, 0, 0, 0, 0]  block_version=9.1.01
  Mult1 : xbsIndex_r4/Mult  precision=Full  arith_type="Signed  (2's comp)"  n_bits=8  bin_pt=2  quantization=Truncate  overflow=Wrap  en=off  latency=mult_latency  dbl_ovrd=off  use_behavioral_HDL=on  opt=Speed  use_embedded=off  optimum_pipeline=off  pipeline=on  use_rpm=on  placement_style=Rectangular shape  block_type=mult
      settings: infoedit=Hardware notes: To use the internal pipeline stage of the dedicated multiplier you must select 'Pipeline for maximum performance'.  xl_area=[0, 0, 0, 0, 0, 0, 0]  block_version=9.1.01
  Reinterpret : xbsIndex_r4/Reinterpret  force_arith_type=on  arith_type="Signed  (2's comp)"  force_bin_pt=on  bin_pt=coeff_frac_width  block_type=reinterpret
      settings: infoedit="Changes signal type without altering the binary representation.   You can changed the signal between signed and unsigned, and relocate the binary point.<P><P>Hardware notes: In hardware this block costs nothing.<P><P>Example:  Suppose the input is 6 bits wide, signed, with 2 fractional bits, and the output is forced to unsigned with 0 fractional bits.  Then an input of -2.0 (1110.00 in binary 2's complement) becomes an output of 56 (111000 in binary)."  block_version=9.1.01
  Slice : xbsIndex_r4/Slice  nbits=coeff_width  boolean_output=off  mode=Lower Bit Location + Width  bit1=0  base1=MSB of Input  bit0=0  base0=LSB of Input  dbl_ovrd=off  block_type=slice
      settings: infoedit="Extracts a given range of bits from each input sample and presents it at the output.  The output type is ordinarily unsigned with binary point at zero, but can be Boolean when the slice is one bit wide.<P><P>Hardware notes: In hardware this block costs nothing."  block_version=9.1.01
  Slice1 : xbsIndex_r4/Slice  nbits=0  boolean_output=off  mode=Two Bit Locations  bit1=0  base1=MSB of Input  bit0=coeff_width  base0=LSB of Input  dbl_ovrd=off  block_type=slice
      settings: infoedit="Extracts a given range of bits from each input sample and presents it at the output.  The output type is ordinarily unsigned with binary point at zero, but can be Boolean when the slice is one bit wide.<P><P>Hardware notes: In hardware this block costs nothing."  block_version=9.1.01
  c_to_ri : casper_library_misc/c_to_ri  SystemSampleTime=-1  n_bits=data_width  bin_pt=data_width-1
      settings: AttributesFormatString=12_11 r/i
  delay_bram : casper_library_delays/delay_bram  SystemSampleTime=-1  DelayLen=delay  bram_latency=bram_latency  use_dsp48=off
  ri_to_c : Subsystem
  sync_delay : casper_library_delays/sync_delay  SystemSampleTime=-1  DelayLen=delay
  dout : Outport  OutDataType=sfix(16)  OutScaling=2^0
  sync_out : Outport  Port=2  OutDataType=sfix(16)  OutScaling=2^0
  coeff_out : Outport  Port=3  OutDataType=sfix(16)  OutScaling=2^0
  taps_out : Outport  Port=4  OutDataType=sfix(16)  OutScaling=2^0
  wires:
  delay_bram/1 -> dout/1
  din/1 -> delay_bram/1, c_to_ri/1
  c_to_ri/2 -> Mult/1
  c_to_ri/1 -> Mult1/1
  ri_to_c/1(c) -> Concat/1
  Mult/1 -> ri_to_c/2(im)
  Mult1/1 -> ri_to_c/1(re)
  sync/1 -> sync_delay/1
  sync_delay/1 -> sync_out/1
  taps/1 -> Concat/2
  Concat/1 -> taps_out/1
  coeff/1 -> Slice/1, Slice1/1
  Slice1/1 -> coeff_out/1
  Slice/1 -> Reinterpret/1
  Reinterpret/1 -> Mult1/2, Mult/2

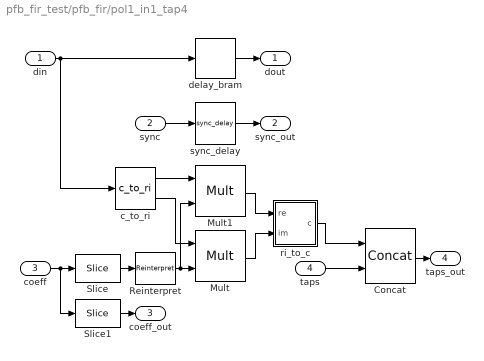
== system pfb_fir_test/pfb_fir/pol1_in1_tap4 ==
  din : Inport  OutDataType=sfix(16)  OutScaling=2^0
  sync : Inport  Port=2  OutDataType=sfix(16)  OutScaling=2^0
  coeff : Inport  Port=3  OutDataType=sfix(16)  OutScaling=2^0
  taps : Inport  Port=4  OutDataType=sfix(16)  OutScaling=2^0
  Concat : xbsIndex_r4/Concat  num_inputs=2  dbl_ovrd=off  block_type=concat
      settings: block_version=9.1.01
  Mult : xbsIndex_r4/Mult  precision=Full  arith_type="Signed  (2's comp)"  n_bits=8  bin_pt=2  quantization=Truncate  overflow=Wrap  en=off  latency=mult_latency  dbl_ovrd=off  use_behavioral_HDL=on  opt=Speed  use_embedded=off  optimum_pipeline=off  pipeline=on  use_rpm=on  placement_style=Rectangular shape  block_type=mult
      settings: infoedit=Hardware notes: To use the internal pipeline stage of the dedicated multiplier you must select 'Pipeline for maximum performance'.  xl_area=[0, 0, 0, 0, 0, 0, 0]  block_version=9.1.01
  Mult1 : xbsIndex_r4/Mult  precision=Full  arith_type="Signed  (2's comp)"  n_bits=8  bin_pt=2  quantization=Truncate  overflow=Wrap  en=off  latency=mult_latency  dbl_ovrd=off  use_behavioral_HDL=on  opt=Speed  use_embedded=off  optimum_pipeline=off  pipeline=on  use_rpm=on  placement_style=Rectangular shape  block_type=mult
      settings: infoedit=Hardware notes: To use the internal pipeline stage of the dedicated multiplier you must select 'Pipeline for maximum performance'.  xl_area=[0, 0, 0, 0, 0, 0, 0]  block_version=9.1.01
  Reinterpret : xbsIndex_r4/Reinterpret  force_arith_type=on  arith_type="Signed  (2's comp)"  force_bin_pt=on  bin_pt=coeff_frac_width  block_type=reinterpret
      settings: infoedit="Changes signal type without altering the binary representation.   You can changed the signal between signed and unsigned, and relocate the binary point.<P><P>Hardware notes: In hardware this block costs nothing.<P><P>Example:  Suppose the input is 6 bits wide, signed, with 2 fractional bits, and the output is forced to unsigned with 0 fractional bits.  Then an input of -2.0 (1110.00 in binary 2's complement) becomes an output of 56 (111000 in binary)."  block_version=9.1.01
  Slice : xbsIndex_r4/Slice  nbits=coeff_width  boolean_output=off  mode=Lower Bit Location + Width  bit1=0  base1=MSB of Input  bit0=0  base0=LSB of Input  dbl_ovrd=off  block_type=slice
      settings: infoedit="Extracts a given range of bits from each input sample and presents it at the output.  The output type is ordinarily unsigned with binary point at zero, but can be Boolean when the slice is one bit wide.<P><P>Hardware notes: In hardware this block costs nothing."  block_version=9.1.01
  Slice1 : xbsIndex_r4/Slice  nbits=0  boolean_output=off  mode=Two Bit Locations  bit1=0  base1=MSB of Input  bit0=coeff_width  base0=LSB of Input  dbl_ovrd=off  block_type=slice
      settings: infoedit="Extracts a given range of bits from each input sample and presents it at the output.  The output type is ordinarily unsigned with binary point at zero, but can be Boolean when the slice is one bit wide.<P><P>Hardware notes: In hardware this block costs nothing."  block_version=9.1.01
  c_to_ri : casper_library_misc/c_to_ri  SystemSampleTime=-1  n_bits=data_width  bin_pt=data_width-1
      settings: AttributesFormatString=12_11 r/i
  delay_bram : casper_library_delays/delay_bram  SystemSampleTime=-1  DelayLen=delay  bram_latency=bram_latency  use_dsp48=off
  ri_to_c : Subsystem
  sync_delay : casper_library_delays/sync_delay  SystemSampleTime=-1  DelayLen=delay
  dout : Outport  OutDataType=sfix(16)  OutScaling=2^0
  sync_out : Outport  Port=2  OutDataType=sfix(16)  OutScaling=2^0
  coeff_out : Outport  Port=3  OutDataType=sfix(16)  OutScaling=2^0
  taps_out : Outport  Port=4  OutDataType=sfix(16)  OutScaling=2^0
  wires:
  delay_bram/1 -> dout/1
  din/1 -> delay_bram/1, c_to_ri/1
  c_to_ri/2 -> Mult/1
  c_to_ri/1 -> Mult1/1
  ri_to_c/1(c) -> Concat/1
  Mult/1 -> ri_to_c/2(im)
  Mult1/1 -> ri_to_c/1(re)
  sync/1 -> sync_delay/1
  sync_delay/1 -> sync_out/1
  taps/1 -> Concat/2
  Concat/1 -> taps_out/1
  coeff/1 -> Slice/1, Slice1/1
  Slice1/1 -> coeff_out/1
  Slice/1 -> Reinterpret/1
  Reinterpret/1 -> Mult1/2, Mult/2
